simulink model "FOC"  (R2024b)
settings: Solver=VariableStepAuto  StartTime=0.0  StopTime=0.4  FixedStep=0.0001  RelTol=1e-3
values from neighbouring files (symbols this model uses):
  fc = 1000000    [data.m]
  flux = 0.005753    [data.m]
  fsp = 100000    [data.m]
  J = 0.00002    (= 2e-05)    [data.m]
  Ki_c = R * Wc    (= 3769911.18431)    [data.m]
  Ki_s = Kp_s * (Wsp / 5)    (= 45748209.7507)    [data.m]
  Kp_c_d = Ld * Wc    [data.m]
  Kp_c_q = Lq * Wc    (= 3518.58377202)    [data.m]
  Kp_s = (J * Wsp) / (1.5 * Pn * flux)    (= 364.052685971)    [data.m]
  Lq = 0.00056    [data.m]
  Pn = 4    [data.m]
  R = 0.6    [data.m]
  Ts = 1e-06    [data.m]
undefined symbols (not defined in the file or in its folder): DiscIntNeverNeededParam, Ld, PI
libraries: powerlib_extras x2, simulink x2, spsDCVoltageSourceLib x1, spsPermanentMagnetSynchronousMachineLib x1, slpidlib x1, spsUniversalBridgeLib x1, spspowerguiLib x1
settings Model: Creator=TUMI  LastModifiedBy=23768
settings OptimizationCC: ReuseModelBlockBuffer=off
settings RTWCC: GPUComputeCapability=3.5

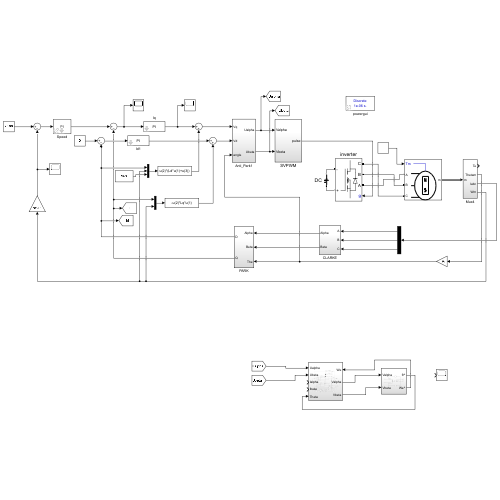
[thumbnail: Simulink's stored preview of the top-level diagram]
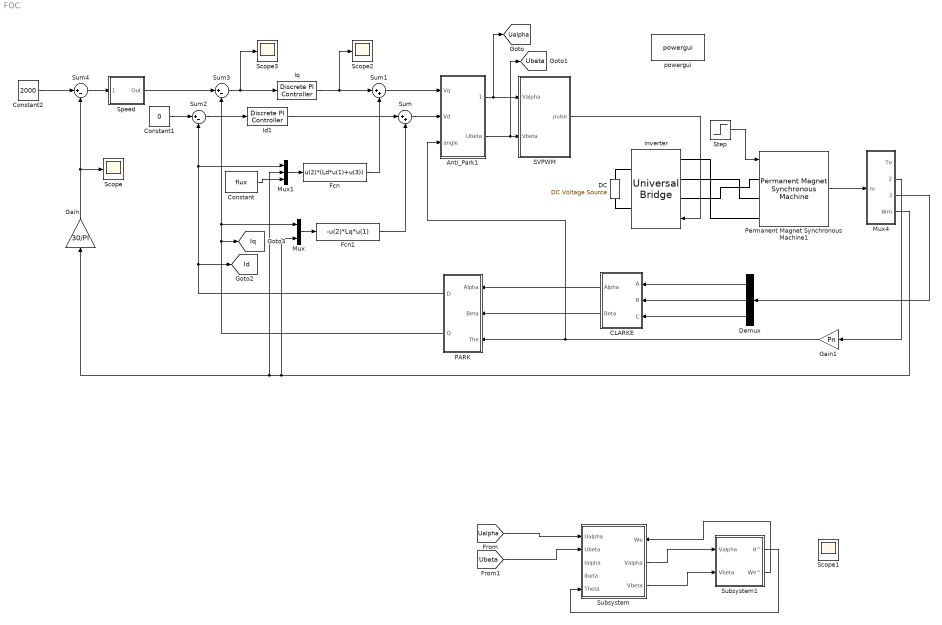
== system FOC ==
  Anti_Park1 : Subsystem
  CLARKE : Subsystem
  Constant : Constant  Value=flux
  Constant1 : Constant  Value=0
  Constant2 : Constant  Value=2000
  DC : spsDCVoltageSourceLib/DC Voltage Source  Amplitude=24  Measurements=Voltage
  Demux : Demux  Outputs=3
  Fcn : Fcn  Expr=u(2)*(Ld*u(1)+u(3))
  Fcn1 : Fcn  Expr=-u(2)*Lq*u(1)
  Gain : Gain  Gain=30/PI
  Gain1 : Gain  Gain=Pn
  Id1 : powerlib_extras/Discrete  Control Blocks/Discrete PI Controller  Kp=Kp_c_d  Ki=Ki_c  Par_Limits=[24*0.9*sqrt(1/3) -24*0.9*sqrt(1/3)]  Init=0  Ts=1/fc
  Iq : powerlib_extras/Discrete  Control Blocks/Discrete PI Controller  Kp=Kp_c_q  Ki=Ki_c  Par_Limits=[24*0.9*sqrt(1/3) -24*0.9*sqrt(1/3)]  Init=0  Ts=1/fc
  Mux : Mux  Inputs=2
  Mux1 : Mux  Inputs=3
  Mux4 : Subsystem
  PARK : Subsystem
  Permanent Magnet Synchronous Machine1 : spsPermanentMagnetSynchronousMachineLib/Permanent Magnet Synchronous Machine  NbPhases=3  FluxDistribution=Sinusoidal  RotorType=Round  MechanicalLoad=Torque Tm  PresetModel=No  ShowDetailedParameters=on  MeasurementBus=off  Resistance=0.6  Inductance=0  dqInductances=[Ld,Lq]  La=[0.000279]  MachineConstant=Voltage Constant (V_peak L-L / krpm)  Flux=0.00572  VoltageCst=4.15  TorqueCst=0.03432  Flat=0  Mechanical=[J,1e-5,Pn,0]  PolePairs=4  InitialConditions=[0,0,0,0]  InitialConditions5ph=[0 0 0 0 0 0]  RefAngle=Aligned with phase A axis (original Park)  IterativeDiscreteModel=Trapezoidal non iterative  TsBlock=-1  TsPowergui=0
      link override From: GotoTag=T47_4340_3633560483959
      settings: AttributesFormatString=\n
  SVPWM : Subsystem
  Scope{,1..3} (4 alike) : Scope
  Speed : Subsystem  AncestorBlock=|  DialogController=POWERSYS.PowerSysDialog  mask(Discrete PI Controller){Kp=Kp_s, Ki=Ki_s, Par_Limits=[100,-100], Init=0, Ts=1/fsp}
      | powerlib_extras/Discrete 
      | Control Blocks/Discrete
      | PI Controller
      mask prompts: Kp "Proportional gain (Kp):"; Ki "Integral gain (Ki):"; Par_Limits "Output limits: [ Upper   Lower ]"; Init "Output initial value:"; Ts "Sample time:"
      mask help: This block implements a discrete PI controller.
      mask init:
      | UpperLimit=Par_Limits(1);
      | LowerLimit=Par_Limits(2);
      | power_initmask();
      settings: LibrarySourceBlock=|
      | powerlib_extras/Discrete
      | Control Blocks/Discrete
      | PI Controller
      mask Help: This block is part of a subset of blocks in the Extras library that does not have documentation associated with it, other than the block mask description.
      mask Display: disp('PI');
  Step : Step  Time=0.2  After=0  SampleTime=0
  Subsystem : Subsystem
      settings: PortSchema="{\"entries\":[{\"content\":{\"sides\":[{\"content\":{\"connectorIds\":[\"In1\",\"In2\",\"In3\",\"In4\",\"In5\"]},\"type\":\"ConnectorPlacement.EquallySpacedRectSide\",\"uuid\":\"aced71a6-c066-4fc9-99bb-f6855d87aa3e\"},{\"content\":{\"connectorIds\":[\"In6\",\"Out1\",\"Out2\"],\"side\":\"RIGHT\"},\"type\":\"ConnectorPlacement.EquallySpacedRectSide\",\"uuid\":\"6d40580d-0945-4a65-9035-c3ecbdbde77f\"},{\"content\":{\"connectorIds\":[],\"side\":\"TOP\"},\"type\":\"ConnectorPlacement.EquallySpacedRectSide\",\"uuid\":\"d41dcef0-52e7-4575-84ca-0c4ef03a7588\"}]},\"type\":\"ConnectorPlacement.EquallySpacedConnector\",\"uuid\":\"77d8cb2d-ec4b-4f93-952a-2798ef7d3ecc\"}],\"packageUris\":[\"http://schema.mathworks.com/mf0/Connector/R2020b\"],\"version\":\"1.0\"}"
  Subsystem1 : Subsystem
  Sum : Sum  Inputs=|++
  Sum1 : Sum  Inputs=|++
  Sum2 : Sum  Inputs=|+-
  Sum3 : Sum  Inputs=|+-
  Sum4 : Sum  Inputs=|+-
  inverter : spsUniversalBridgeLib/Universal Bridge  Arms=3  SnubberResistance=100  SnubberCapacitance=1e-5  Device=MOSFET / Diodes  Ron=1e-3  Lon=0  ForwardVoltages="[  0  0  ]"  ForwardVoltage=0  GTOparameters=[ 10e-6 , 20e-6 ]  IGBTparameters=[ 1e-6 , 2e-6 ]  Measurements=None  Measurements_2=None  converterType=Rectifier
  powergui : spspowerguiLib/powergui  Priority=1  SimulationMode=Discrete  SampleTime=Ts  frequency=60  Iterations=50  frequencyindice=0  Pbase=100e6  ErrMax=1e-4  UnitsV=kV  UnitsW=MW  buscounter=0  FunctionMessages=off  echomessages=off  EnableUseOfTLC=off  CurrentSourceSwitches=off  DisableSnubberDevices=off  DisableRonSwitches=off  DisableVfSwitches=off  DisplayEquations=off  AutomaticDiscreteSolvers=off  SolverType=Tustin/Backward Euler (TBE)  Interpol=off  ExternalGateDelay=off  methode=off  Ts=100  x0status=blocks  SPID=on  SwTol=0  HookPort=off  NonlinearTolerance=1e-4  nMaxIteration=100  ContinueOnMaxIteration=off  RestoreLinks=warning  ResistiveCurrentMeasurement=off  Frange=[0:2:500]  Ylog=off  Xlog=on  ShowGrid=off  save=off  variable=ZData  structure=0  ZoomFFT=off  StartTime=0.0  cycles=1  DisplayStyle=1  fundamental=60  FreqAxis=off  MaxFrequency=1000  frequencyindicesteady=1  RmsSteady=1  display=off
  tag scope: Id=global, Iq=global, Ualpha=global, Ubeta=global
  wires:
  CLARKE/2(Beta) -> PARK/2(Beta)
  CLARKE/1(Alpha) -> PARK/1(Alpha)
  Demux/3 -> CLARKE/3(C)
  Demux/2 -> CLARKE/2(B)
  Demux/1 -> CLARKE/1(A)
  Mux4/3(Iabc) -> Demux/1
  Permanent Magnet Synchronous Machine1/1 -> Mux4/1(m)
  Anti_Park1/2(Ubeta) -> [Ubeta], SVPWM/2(Vbeta)
  Anti_Park1/1(Ualpha) -> [Ualpha], SVPWM/1(Valpha)
  SVPWM/1(pulse) -> inverter/1
  Iq/1 -> Scope2/1, Sum1/1
  Sum1/1 -> Anti_Park1/1(Vq)
  Sum/1 -> Anti_Park1/2(Vd)
  Id1/1 -> Sum/1
  PARK/1(D) -> [Id], Sum2/2, Mux1/1
  Constant1/1 -> Sum2/1
  Sum2/1 -> Id1/1
  Sum3/1 -> Scope3/1, Iq/1
  PARK/2(Q) -> [Iq], Mux/1, Sum3/2
  Mux1/1 -> Fcn/1
  Mux/1 -> Fcn1/1
  Fcn1/1 -> Sum/2
  Constant/1 -> Mux1/3
  Speed/1(Out) -> Sum3/1
  Sum4/1 -> Speed/1(Error)
  Gain/1 -> Scope/1, Sum4/2
  Fcn/1 -> Sum1/2
  [Ualpha] -> Subsystem/1(Ualpha)
  [Ubeta] -> Subsystem/2(Ubeta)
  Subsystem/1(Valpha) -> Subsystem1/1(Valpha)
  Subsystem/2(Vbeta) -> Subsystem1/2(Vbeta)
  Subsystem1/1(θ^) -> Subsystem/5(Theta)
  Step/1 -> Permanent Magnet Synchronous Machine1/1
  Mux4/4(Wm) -> Gain/1, Mux1/2, Mux/2
  Subsystem1/2(We^) -> Subsystem/6(We)
  Mux4/2(Thetam) -> Gain1/1
  Gain1/1 -> PARK/3(The), Anti_Park1/3(angle)
  Constant2/1 -> Sum4/1
  connections:
  DC/LConn1 -- inverter/RConn2
  DC/RConn1 -- inverter/RConn1
  inverter/LConn1 -- Permanent Magnet Synchronous Machine1/LConn1
  inverter/LConn2 -- Permanent Magnet Synchronous Machine1/LConn2
  inverter/LConn3 -- Permanent Magnet Synchronous Machine1/LConn3

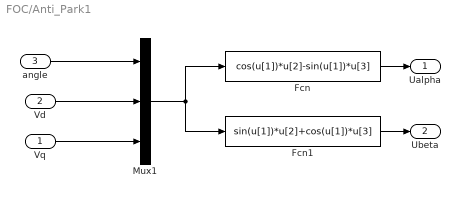
== system FOC/Anti_Park1 ==
  Vq : Inport
  Vd : Inport  Port=2
  angle : Inport  Port=3
  Fcn : Fcn  Expr=cos(u[1])*u[2]-sin(u[1])*u[3]
  Fcn1 : Fcn  Expr=sin(u[1])*u[2]+cos(u[1])*u[3]
  Mux1 : Mux  Inputs=3
  Ualpha : Outport
  Ubeta : Outport  Port=2
  wires:
  Fcn1/1 -> Ubeta/1
  Fcn/1 -> Ualpha/1
  Mux1/1 -> Fcn/1, Fcn1/1
  Vd/1 -> Mux1/2
  Vq/1 -> Mux1/3
  angle/1 -> Mux1/1

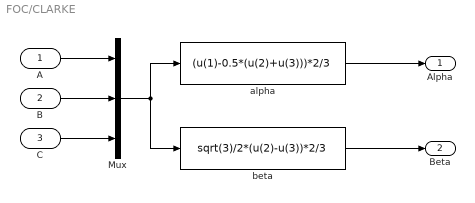
== system FOC/CLARKE ==
  A : Inport
  B : Inport  Port=2
  C : Inport  Port=3
  Mux : Mux  Inputs=3
  alpha : Fcn  Expr=(u(1)-0.5*(u(2)+u(3)))*2/3
  beta : Fcn  Expr=sqrt(3)/2*(u(2)-u(3))*2/3
  Alpha : Outport
  Beta : Outport  Port=2
  wires:
  alpha/1 -> Alpha/1
  B/1 -> Mux/2
  C/1 -> Mux/3
  A/1 -> Mux/1
  Mux/1 -> beta/1, alpha/1
  beta/1 -> Beta/1

== system FOC/Mux4 ==
  m : Inport
  Bus Selector : BusSelector  OutputSignals=Stator current is_a (A),Stator current is_b (A),Stator current is_c (A)
  Bus Selector1 : BusSelector  OutputSignals=Rotor speed wm (rad/s),Rotor angle thetam (rad),Electromagnetic torque Te (N*m)
  Mux : Mux  Inputs=3
  Te : Outport
  Thetam : Outport  Port=2
  Iabc : Outport  Port=3
  Wm : Outport  Port=4
  wires:
  Mux/1 -> Iabc/1
  Bus Selector/1 -> Mux/1  "<Stator current is_a (A)>"
  Bus Selector/3 -> Mux/3  "<Stator current is_c (A)>"
  Bus Selector/2 -> Mux/2  "<Stator current is_b (A)>"
  m/1 -> Bus Selector1/1, Bus Selector/1
  Bus Selector1/3 -> Te/1  "<Electromagnetic torque Te (N*m)>"
  Bus Selector1/2 -> Thetam/1  "<Rotor angle thetam (rad)>"
  Bus Selector1/1 -> Wm/1  "<Rotor speed wm (rad/s)>"

== system FOC/PARK ==
  Alpha : Inport
  Beta : Inport  Port=2
  The : Inport  Port=3
  Mux : Mux  Inputs=3
  d : Fcn  Expr=u(1)*cos(u(3))+u(2)*sin(u(3))
  q : Fcn  Expr=-u(1)*sin(u(3))+u(2)*cos(u(3))
  D : Outport
  Q : Outport  Port=2
  wires:
  d/1 -> D/1
  Beta/1 -> Mux/2
  Alpha/1 -> Mux/1
  Mux/1 -> q/1, d/1
  q/1 -> Q/1
  The/1 -> Mux/3

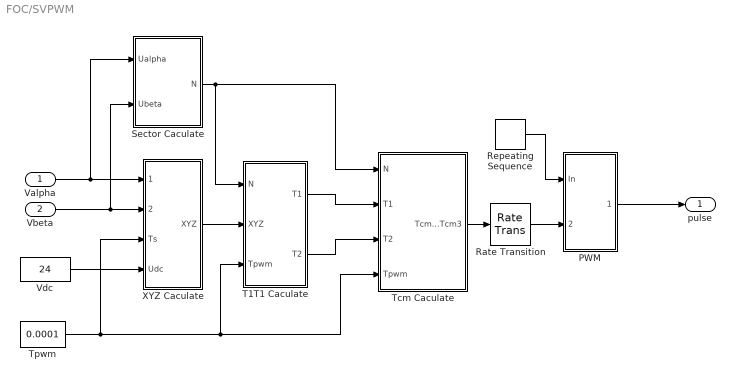
== system FOC/SVPWM ==
  Valpha : Inport
  Vbeta : Inport  Port=2
  PWM : Subsystem
  Rate Transition : RateTransition  OutPortSampleTime=1e-6
  Repeating Sequence : simulink/Sources/Repeating Sequence  rep_seq_t=[0 0.00005 0.0001]  rep_seq_y=[0 0.00005 0]
  Sector Caculate : Subsystem
  T1T1 Caculate : Subsystem
  Tcm Caculate : Subsystem
  Tpwm : Constant  Value=0.0001
  Vdc : Constant  Value=24
  XYZ Caculate : Subsystem
  pulse : Outport
  wires:
  PWM/1(PWM) -> pulse/1
  Repeating Sequence/1 -> PWM/1(In)
  Vbeta/1 -> XYZ Caculate/2(Ubeta), Sector Caculate/2(Ubeta)
  T1T1 Caculate/1(T1) -> Tcm Caculate/2(T1)
  Valpha/1 -> XYZ Caculate/1(Ualpha), Sector Caculate/1(Ualpha)
  T1T1 Caculate/2(T2) -> Tcm Caculate/3(T2)
  Sector Caculate/1("N ") -> Tcm Caculate/1(N), T1T1 Caculate/1(N)
  XYZ Caculate/1(XYZ) -> T1T1 Caculate/2(XYZ)
  Tpwm/1 -> XYZ Caculate/3(Ts), Tcm Caculate/4(Tpwm), T1T1 Caculate/3(Tpwm)
  Vdc/1 -> XYZ Caculate/4(Udc)
  Tcm Caculate/1(Tcm1 Tcm2 Tcm3) -> Rate Transition/1
  Rate Transition/1 -> PWM/2(Tcm123)

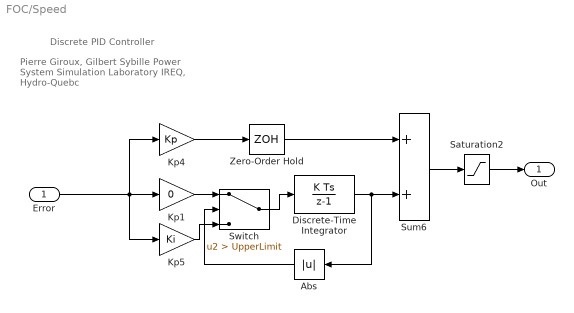
== system FOC/Speed ==
  note: Discrete PID Controller
  note: Pierre Giroux, Gilbert Sybille
      | Power System Simulation Laboratory
      | IREQ, Hydro-Quebc
  Error : Inport  SampleTime=Ts
  Abs : Abs  SaturateOnIntegerOverflow=off
  Discrete-Time Integrator : DiscreteIntegrator  InitialCondition=Init  SampleTime=Ts  LimitOutput=on  UpperSaturationLimit=UpperLimit  LowerSaturationLimit=LowerLimit  ICPrevOutput=DiscIntNeverNeededParam  ICPrevScaledInput=DiscIntNeverNeededParam
  Kp1 : Gain  Gain=0  SaturateOnIntegerOverflow=on  SampleTime=Ts  OutDataTypeStr=Inherit: Same as input  ParamDataTypeStr=Inherit: Same as input
  Kp4 : Gain  Gain=Kp  SaturateOnIntegerOverflow=on  SampleTime=Ts  OutDataTypeStr=Inherit: Same as input  ParamDataTypeStr=Inherit: Same as input
  Kp5 : Gain  Gain=Ki  SaturateOnIntegerOverflow=on  SampleTime=Ts  OutDataTypeStr=Inherit: Same as input  ParamDataTypeStr=Inherit: Same as input
  Saturation2 : Saturate  UpperLimit=UpperLimit  LowerLimit=LowerLimit  SampleTime=Ts
  Sum6 : Sum  InputSameDT=on  SaturateOnIntegerOverflow=on  SampleTime=Ts  OutDataTypeStr=Inherit: Same as first input
  Switch : Switch  Criteria=u2 > Threshold  Threshold=UpperLimit  SaturateOnIntegerOverflow=off  InputSameDT=off
  Zero-Order Hold : ZeroOrderHold  SampleTime=Ts
  Out : Outport  SampleTime=Ts  InitialOutput=0  VectorParamsAs1DForOutWhenUnconnected=off
  wires:
  Zero-Order Hold/1 -> Sum6/1
  Saturation2/1 -> Out/1
  Discrete-Time Integrator/1 -> Abs/1, Sum6/2
  Kp4/1 -> Zero-Order Hold/1
  Sum6/1 -> Saturation2/1
  Error/1 -> Kp4/1, Kp1/1, Kp5/1
  Switch/1 -> Discrete-Time Integrator/1
  Abs/1 -> Switch/2
  Kp5/1 -> Switch/3
  Kp1/1 -> Switch/1

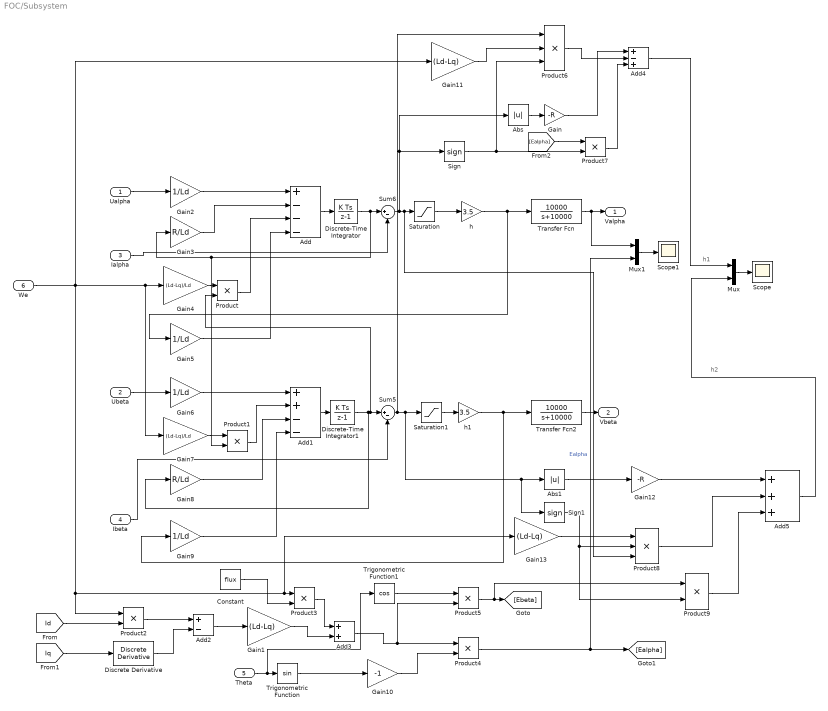
== system FOC/Subsystem ==
  note: h2
  note: h1
  Ualpha : Inport
  Ubeta : Inport  Port=2
  Ialpha : Inport  Port=3
  Ibeta : Inport  Port=4
  Theta : Inport  Port=5
  We : Inport  Port=6
  Abs : Abs  SaturateOnIntegerOverflow=off
  Abs1 : Abs  SaturateOnIntegerOverflow=off
  Add : Sum  Inputs=+---
  Add1 : Sum  Inputs=++--
  Add2 : Sum  Inputs=+-
  Add3 : Sum
  Add4 : Sum  Inputs=+-+
  Add5 : Sum  Inputs=+++
  Constant : Constant  Value=flux
  Discrete Derivative : simulink/Discrete/Discrete Derivative  gainval=1.0  ICPrevScaledInput=0.0  OutMin=[]  OutMax=[]  OutDataType=fixdt(1, 16)  OutScaling=2^-10  DoSatur=off
  Discrete-Time Integrator : DiscreteIntegrator  SampleTime=5e-06  ICPrevOutput=DiscIntNeverNeededParam  ICPrevScaledInput=DiscIntNeverNeededParam
  Discrete-Time Integrator1 : DiscreteIntegrator  SampleTime=5e-06  ICPrevOutput=DiscIntNeverNeededParam  ICPrevScaledInput=DiscIntNeverNeededParam
  Gain : Gain  Gain=-R
  Gain1 : Gain  Gain=(Ld-Lq)
  Gain10 : Gain  Gain=-1
  Gain11 : Gain  Gain=(Ld-Lq)
  Gain12 : Gain  Gain=-R
  Gain13 : Gain  Gain=(Ld-Lq)
  Gain{2,5..6,9} (4 alike) : Gain  Gain=1/Ld
  Gain3 : Gain  Gain=R/Ld
  Gain4 : Gain  Gain=(Ld-Lq)/Ld
  Gain7 : Gain  Gain=(Ld-Lq)/Ld
  Gain8 : Gain  Gain=R/Ld
  Mux : Mux  Inputs=2
  Mux1 : Mux  Inputs=2
  Product{,1..5,7,9} (8 alike) : Product
  Product6 : Product  Inputs=3
  Product8 : Product  Inputs=3
  Saturation : Saturate  UpperLimit=1.0  LowerLimit=-1.0
  Saturation1 : Saturate  UpperLimit=1.0  LowerLimit=-1.0
  Scope : Scope
  Scope1 : Scope
  Sign : Signum
  Sign1 : Signum
  Sum5 : Sum  Inputs=|+-
  Sum6 : Sum  Inputs=|+-
  Transfer Fcn : TransferFcn  Numerator=[10000]  Denominator=[1 10000]
  Transfer Fcn2 : TransferFcn  Numerator=[10000]  Denominator=[1 10000]
  Trigonometric Function : Trigonometry
  Trigonometric Function1 : Trigonometry  Operator=cos
  h : Gain  Gain=3.5
  h1 : Gain  Gain=3.5
  Valpha : Outport
  Vbeta : Outport  Port=2
  wires:
  Ibeta/1 -> Sum5/2
  Sum6/1 -> Sign/1, Abs/1, Product8/3, Saturation/1
  h1/1 -> Transfer Fcn2/1, Gain9/1
  Discrete-Time Integrator1/1 -> Sum5/1, Product/2, Gain8/1
  Saturation/1 -> h/1
  Product1/1 -> Add1/2
  h/1 -> Transfer Fcn/1, Gain5/1
  Gain4/1 -> Product/1
  Discrete-Time Integrator/1 -> Sum6/1, Product1/2, Gain3/1
  Gain2/1 -> Add/1
  We/1 -> Gain11/1, Product3/1, Gain13/1, Product2/1, Gain7/1, Gain4/1
  Sum5/1 -> Sign1/1, Abs1/1, Saturation1/1, Product6/1
  Ualpha/1 -> Gain2/1
  Add/1 -> Discrete-Time Integrator/1
  Gain5/1 -> Add/4
  Add1/1 -> Discrete-Time Integrator1/1
  Gain3/1 -> Add/2
  Saturation1/1 -> h1/1
  Gain6/1 -> Add1/1
  Ubeta/1 -> Gain6/1
  Gain7/1 -> Product1/1
  Product/1 -> Add/3
  Gain9/1 -> Add1/4
  Gain8/1 -> Add1/3
  Ialpha/1 -> Sum6/2
  Transfer Fcn/1 -> Mux1/1, Valpha/1
  Transfer Fcn2/1 -> Vbeta/1
  [Id] -> Product2/2
  Product2/1 -> Add2/1
  [Iq] -> Discrete Derivative/1
  Discrete Derivative/1 -> Add2/2
  Add2/1 -> Gain1/1
  Product3/1 -> Add3/1
  Gain1/1 -> Add3/2
  Constant/1 -> Product3/2
  Trigonometric Function/1 -> Gain10/1
  Theta/1 -> Trigonometric Function1/1, Trigonometric Function/1
  Gain10/1 -> Product4/2
  Add3/1 -> Product5/2, Product4/1
  Trigonometric Function1/1 -> Product5/1
  Abs/1 -> Gain/1
  Gain11/1 -> Product6/2
  Sign/1 -> Product6/3, Product7/2
  Gain/1 -> Add4/1
  Product6/1 -> Add4/2
  Product7/1 -> Add4/3
  Product5/1 -> Product9/1, [Ebeta]
  Product4/1 -> Mux1/2, [Ealpha]  "Ealpha"
  [Ealpha] -> Product7/1
  Mux/1 -> Scope/1
  Add4/1 -> Mux/1
  Abs1/1 -> Gain12/1
  Gain12/1 -> Add5/1
  Gain13/1 -> Product8/1
  Product8/1 -> Add5/2
  Product9/1 -> Add5/3
  Add5/1 -> Mux/2
  Sign1/1 -> Product9/2, Product8/2
  Mux1/1 -> Scope1/1

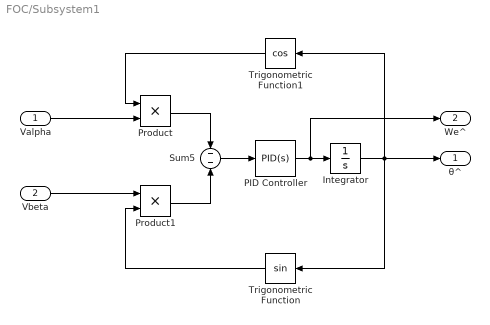
== system FOC/Subsystem1 ==
  Valpha : Inport
  Vbeta : Inport  Port=2
  Integrator : Integrator
  PID Controller : slpidlib/PID Controller  Controller=PID  Form=Parallel  TimeDomain=Continuous-time  UseExternalTs=off  SampleTime=-1  IntegratorMethod=Forward Euler  FilterMethod=Forward Euler  ControllerParametersSource=internal  P=540  I=18000  UseKiTs=off  D=0  UseExternalDerivativeSource=off  N=100  UseFilter=on  TunerSelectOption=Transfer Function Based (PID Tuner App)  InitialConditionSource=internal  InitialConditionForIntegrator=0  InitialConditionForFilter=0  DifferentiatorICPrevScaledInput=0  ExternalReset=none  TrackingMode=off  Kt=1  LimitOutput=off  SatLimitsSource=internal  UpperSaturationLimit=inf  LowerSaturationLimit=-inf  LinearizeAsGain=on  AntiWindupMode=none  Kb=1  LimitIntegrator=off  UpperIntegratorSaturationLimit=inf  LowerIntegratorSaturationLimit=-inf  POutMin=[]  POutMax=[]  IOutMin=[]  IOutMax=[]  DOutMin=[]  DOutMax=[]  NOutMin=[]  NOutMax=[]  SumOutMin=[]  SumOutMax=[]  SaturationOutMin=[]  SaturationOutMax=[]  PParamMin=[]  PParamMax=[]  IParamMin=[]  IParamMax=[]  DParamMin=[]  DParamMax=[]  NParamMin=[]  NParamMax=[]  KbParamMin=[]  KbParamMax=[]  KtParamMin=[]  KtParamMax=[]  KbOutMin=[]  KbOutMax=[]  KtOutMin=[]  KtOutMax=[]  IntegratorOutMin=[]  IntegratorOutMax=[]  FilterOutMin=[]  FilterOutMax=[]  SumI1OutMin=[]  SumI1OutMax=[]  SumI2OutMin=[]  SumI2OutMax=[]  SumI3OutMin=[]  SumI3OutMax=[]  SumI4OutMin=[]  SumI4OutMax=[]  SumDOutMin=[]  SumDOutMax=[]  DifferentiatorOutMin=[]  DifferentiatorOutMax=[]  FilterDiffOutCoefMin=[]  FilterDiffOutCoefMax=[]  ReciprocalOutMin=[]  ReciprocalOutMax=[]  SumDenOutMin=[]  SumDenOutMax=[]  SumNumOutMin=[]  SumNumOutMax=[]  DivideOutMin=[]  DivideOutMax=[]  UdiffTsProdOutMin=[]  UdiffTsProdOutMax=[]  NTsProdOutMin=[]  NTsProdOutMax=[]  UintegralTsProdOutMin=[]  UintegralTsProdOutMax=[]  UngainTsProdOutMin=[]  UngainTsProdOutMax=[]  ClampingZeroOutDataTypeStr=Inherit: Inherit via back propagation  ClampingZeroOutMin=[]  ClampingZeroOutMax=[]  FilterDenConstantOutDataTypeStr=Inherit: Inherit via back propagation  FilterDenConstantOutMin=[]  FilterDenConstantOutMax=[]  PCopyOutDataTypeStr=Inherit: Inherit via back propagation  PCopyOutMin=[]  PCopyOutMax=[]  NCopyOutDataTypeStr=Inherit: Inherit via back propagation  NCopyOutMin=[]  NCopyOutMax=[]  IntegratorContinuousStateAttributes=''  IntegratorStateMustResolveToSignalObject=off  IntegratorRTWStateStorageClass=Auto  FilterContinuousStateAttributes=''  FilterStateMustResolveToSignalObject=off  FilterRTWStateStorageClass=Auto  ParallelPVariant=InternalParameters  IdealPVariant=Disabled  IVariant=InternalParameters  DVariant=InternalParameters  IntegratorVariant=Continuous  SatVariant=Disabled  AWVariant=Passthrough  PCopyVariant=Disabled  TRVariant=Disabled  FdbkBlocksVariant=Forward  IdealPFdbkVariant=Disabled  SatFdbkVariant=Disabled  DerivativeFilterVariant=ContFilter  NVariant=InternalParameters  NCopyVariant=Disabled  FilterICVariant=InternalICsFilter  IntegratorICVariant=InternalICs  ExternalResetVariant=Disabled  TRSumVariant=Passthrough  SumFdbkVariant=Disabled  SumVariant=Sum_PID  TsampFilterVariant=InternalTs  TsampNgainVariant=Passthrough  TsampIntegralVariant=Disabled_SignalSpec  ExternalSaturationOutDataTypeStr=Inherit: Same as second input  DerivativeSourceVariant=ErrorSignal  PreIntVariant=InternalPreInt
  Product : Product
  Product1 : Product
  Sum5 : Sum  Inputs=-|-
  Trigonometric Function : Trigonometry
  Trigonometric Function1 : Trigonometry  Operator=cos
  θ^ : Outport
  We^ : Outport  Port=2
  wires:
  Product1/1 -> Sum5/2
  Integrator/1 -> θ^/1, Trigonometric Function/1, Trigonometric Function1/1
  Trigonometric Function1/1 -> Product/1
  PID Controller/1 -> We^/1, Integrator/1
  Product/1 -> Sum5/1
  Trigonometric Function/1 -> Product1/2
  Sum5/1 -> PID Controller/1
  Vbeta/1 -> Product1/1
  Valpha/1 -> Product/2

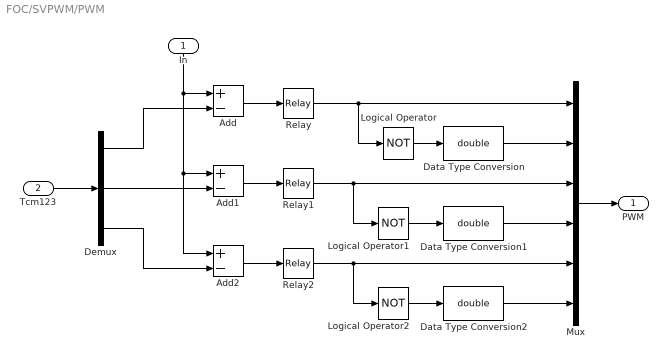
== system FOC/SVPWM/PWM ==
  In : Inport
  Tcm123 : Inport  Port=2
  Add : Sum  Inputs=+-
  Add1 : Sum  Inputs=+-
  Add2 : Sum  Inputs=+-
  Data Type Conversion : DataTypeConversion  OutDataTypeStr=double  SaturateOnIntegerOverflow=off  RndMeth=Floor
  Data Type Conversion1 : DataTypeConversion  OutDataTypeStr=double  SaturateOnIntegerOverflow=off  RndMeth=Floor
  Data Type Conversion2 : DataTypeConversion  OutDataTypeStr=double  SaturateOnIntegerOverflow=off  RndMeth=Floor
  Demux : Demux  Outputs=3
  Logical Operator : Logic  Operator=NOT  AllPortsSameDT=off  OutDataTypeStr=boolean
  Logical Operator1 : Logic  Operator=NOT  AllPortsSameDT=off  OutDataTypeStr=boolean
  Logical Operator2 : Logic  Operator=NOT  AllPortsSameDT=off  OutDataTypeStr=boolean
  Mux : Mux  Inputs=6
  Relay : Relay  OffSwitchValue=-eps
  Relay1 : Relay  OffSwitchValue=-eps
  Relay2 : Relay  OffSwitchValue=-eps
  PWM : Outport
  wires:
  Demux/3 -> Add2/2
  Demux/2 -> Add1/2
  Demux/1 -> Add/2
  Relay2/1 -> Mux/5, Logical Operator2/1
  Relay1/1 -> Mux/3, Logical Operator1/1
  Relay/1 -> Logical Operator/1, Mux/1
  Mux/1 -> PWM/1
  Data Type Conversion/1 -> Mux/2
  Data Type Conversion1/1 -> Mux/4
  Data Type Conversion2/1 -> Mux/6
  Logical Operator2/1 -> Data Type Conversion2/1
  Logical Operator1/1 -> Data Type Conversion1/1
  Logical Operator/1 -> Data Type Conversion/1
  Add1/1 -> Relay1/1
  Add2/1 -> Relay2/1
  Add/1 -> Relay/1
  In/1 -> Add/1, Add2/1, Add1/1
  Tcm123/1 -> Demux/1

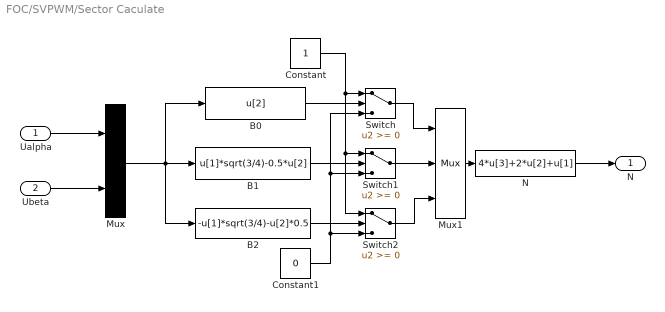
== system FOC/SVPWM/Sector Caculate ==
  Ualpha : Inport
  Ubeta : Inport  Port=2
  B0 : Fcn  Expr=u[2]
  B1 : Fcn  Expr=u[1]*sqrt(3/4)-0.5*u[2]
  B2 : Fcn  Expr=-u[1]*sqrt(3/4)-u[2]*0.5
  Constant : Constant
  Constant1 : Constant  Value=0
  Mux : Mux  Inputs=2
  Mux1 : Mux  Inputs=3
  N : Fcn  Expr=4*u[3]+2*u[2]+u[1]
  Switch : Switch  SaturateOnIntegerOverflow=off  InputSameDT=off
  Switch1 : Switch  SaturateOnIntegerOverflow=off  InputSameDT=off
  Switch2 : Switch  SaturateOnIntegerOverflow=off  InputSameDT=off
  "N " : Outport
  wires:
  Switch2/1 -> Mux1/3
  Switch/1 -> Mux1/1
  Ualpha/1 -> Mux/1
  Ubeta/1 -> Mux/2
  Mux/1 -> B2/1, B1/1, B0/1
  B0/1 -> Switch/2
  B1/1 -> Switch1/2
  B2/1 -> Switch2/2
  Constant/1 -> Switch/1, Switch2/1, Switch1/1
  Constant1/1 -> Switch/3, Switch1/3, Switch2/3
  Switch1/1 -> Mux1/2
  Mux1/1 -> N/1
  N/1 -> "N "/1

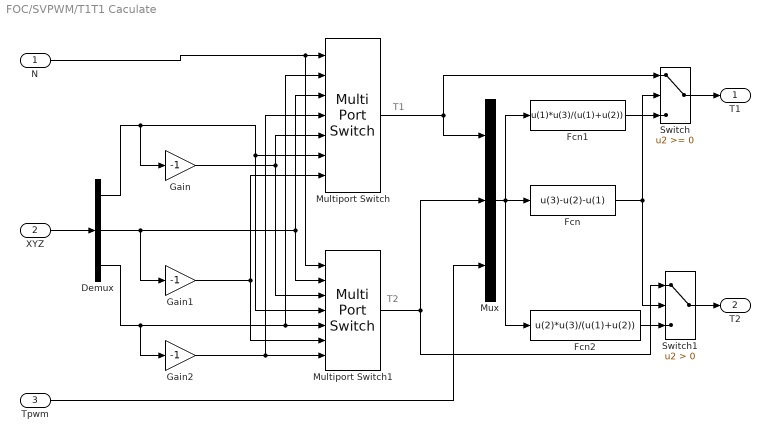
== system FOC/SVPWM/T1T1 Caculate ==
  note: T1
  note: T2
  N : Inport
  XYZ : Inport  Port=2
  Tpwm : Inport  Port=3
  Demux : Demux  Outputs=3
  Fcn : Fcn  Expr=u(3)-u(2)-u(1)
  Fcn1 : Fcn  Expr=u(1)*u(3)/(u(1)+u(2))
  Fcn2 : Fcn  Expr=u(2)*u(3)/(u(1)+u(2))
  Gain : Gain  Gain=-1
  Gain1 : Gain  Gain=-1
  Gain2 : Gain  Gain=-1
  Multiport Switch : MultiPortSwitch  Inputs=6  SaturateOnIntegerOverflow=off  InputSameDT=off
  Multiport Switch1 : MultiPortSwitch  Inputs=6  SaturateOnIntegerOverflow=off  InputSameDT=off
  Mux : Mux  Inputs=3
  Switch : Switch  SaturateOnIntegerOverflow=off  InputSameDT=off
  Switch1 : Switch  Criteria=u2 > Threshold  SaturateOnIntegerOverflow=off  InputSameDT=off
  T1 : Outport
  T2 : Outport  Port=2
  wires:
  Tpwm/1 -> Mux/3
  XYZ/1 -> Demux/1
  Switch1/1 -> T2/1
  Switch/1 -> T1/1
  Fcn2/1 -> Switch1/3
  Fcn1/1 -> Switch/3
  Fcn/1 -> Switch/2, Switch1/2
  Mux/1 -> Fcn1/1, Fcn/1, Fcn2/1
  Multiport Switch/1 -> Switch/1, Mux/1
  Multiport Switch1/1 -> Switch1/1, Mux/2
  N/1 -> Multiport Switch/1, Multiport Switch1/1
  Demux/2 -> Multiport Switch/3, Multiport Switch1/2, Gain1/1
  Demux/3 -> Multiport Switch1/5, Multiport Switch/2, Gain2/1
  Demux/1 -> Multiport Switch/6, Multiport Switch1/4, Gain/1
  Gain/1 -> Multiport Switch1/3, Multiport Switch/5
  Gain2/1 -> Multiport Switch/4, Multiport Switch1/7
  Gain1/1 -> Multiport Switch1/6, Multiport Switch/7

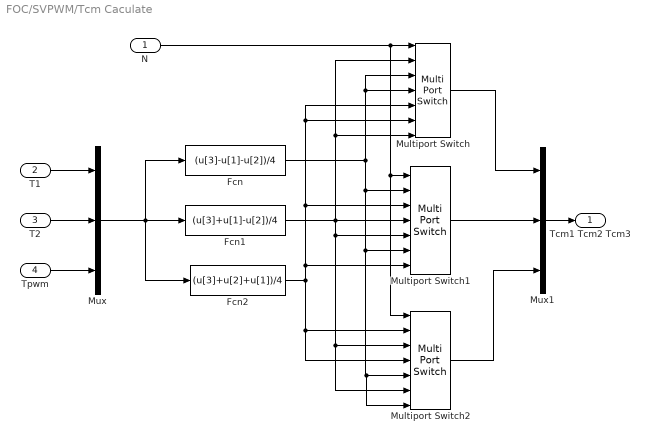
== system FOC/SVPWM/Tcm Caculate ==
  N : Inport
  T1 : Inport  Port=2
  T2 : Inport  Port=3
  Tpwm : Inport  Port=4
  Fcn : Fcn  Expr=(u[3]-u[1]-u[2])/4
  Fcn1 : Fcn  Expr=(u[3]+u[1]-u[2])/4
  Fcn2 : Fcn  Expr=(u[3]+u[2]+u[1])/4
  Multiport Switch : MultiPortSwitch  Inputs=6  SaturateOnIntegerOverflow=off  InputSameDT=off
  Multiport Switch1 : MultiPortSwitch  Inputs=6  SaturateOnIntegerOverflow=off  InputSameDT=off
  Multiport Switch2 : MultiPortSwitch  Inputs=6  SaturateOnIntegerOverflow=off  InputSameDT=off
  Mux : Mux  Inputs=3
  Mux1 : Mux  Inputs=3
  Tcm1 Tcm2 Tcm3 : Outport
  wires:
  Mux/1 -> Fcn2/1, Fcn/1, Fcn1/1
  Tpwm/1 -> Mux/3
  T2/1 -> Mux/2
  T1/1 -> Mux/1
  Multiport Switch2/1 -> Mux1/3
  Multiport Switch1/1 -> Mux1/2
  Multiport Switch/1 -> Mux1/1
  Mux1/1 -> Tcm1 Tcm2 Tcm3/1
  Fcn/1 -> Multiport Switch/3, Multiport Switch/4, Multiport Switch1/6, Multiport Switch2/5, Multiport Switch2/7, Multiport Switch1/2
  Fcn1/1 -> Multiport Switch1/5, Multiport Switch2/3, Multiport Switch2/6, Multiport Switch1/4, Multiport Switch/7, Multiport Switch/2
  Fcn2/1 -> Multiport Switch/5, Multiport Switch/6, Multiport Switch1/3, Multiport Switch1/7, Multiport Switch2/2, Multiport Switch2/4
  N/1 -> Multiport Switch2/1, Multiport Switch1/1, Multiport Switch/1

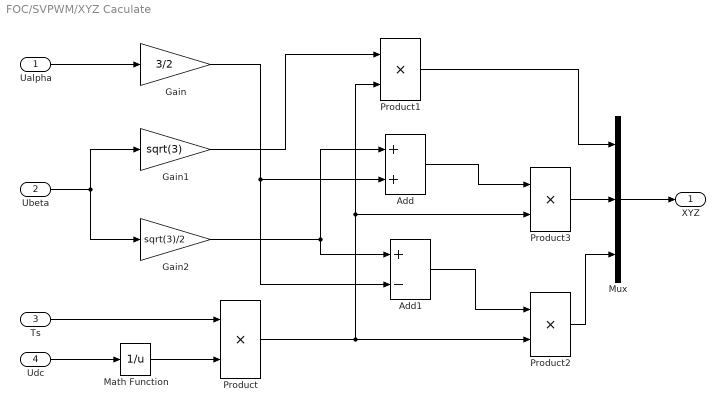
== system FOC/SVPWM/XYZ Caculate ==
  Ualpha : Inport
  Ubeta : Inport  Port=2
  Ts : Inport  Port=3
  Udc : Inport  Port=4
  Add : Sum
  Add1 : Sum  Inputs=+-
  Gain : Gain  Gain=3/2
  Gain1 : Gain  Gain=sqrt(3)
  Gain2 : Gain  Gain=sqrt(3)/2
  Math Function : Math  Operator=reciprocal  SignedPower=on
  Mux : Mux  Inputs=3
  Product{,1..3} (4 alike) : Product  RndMeth=Zero
  XYZ : Outport
  wires:
  Mux/1 -> XYZ/1
  Product1/1 -> Mux/1
  Product3/1 -> Mux/2
  Product2/1 -> Mux/3
  Ualpha/1 -> Gain/1
  Ubeta/1 -> Gain2/1, Gain1/1
  Udc/1 -> Math Function/1
  Math Function/1 -> Product/2
  Ts/1 -> Product/1
  Gain1/1 -> Product1/1
  Product/1 -> Product2/2, Product1/2, Product3/2
  Gain/1 -> Add1/2, Add/2
  Gain2/1 -> Add/1, Add1/1
  Add1/1 -> Product2/1
  Add/1 -> Product3/1
